simulink model "Third_order_loop"  (R2025a)
settings: Solver=VariableStepAuto  StartTime=0.0  StopTime=100  RelTol=1e-3
libraries: simulink x2
settings Model: Creator=庞亚宸  LastModifiedBy=庞亚宸

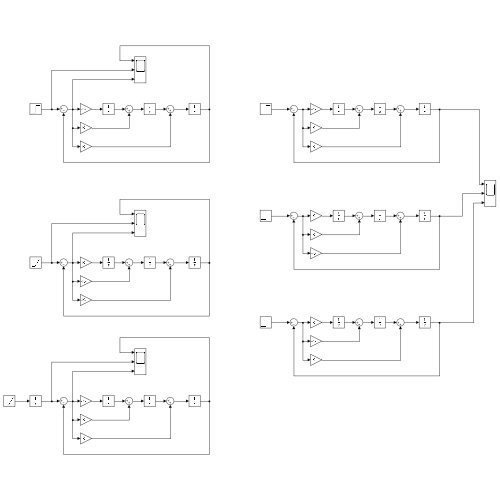
[thumbnail: Simulink's stored preview of the top-level diagram]
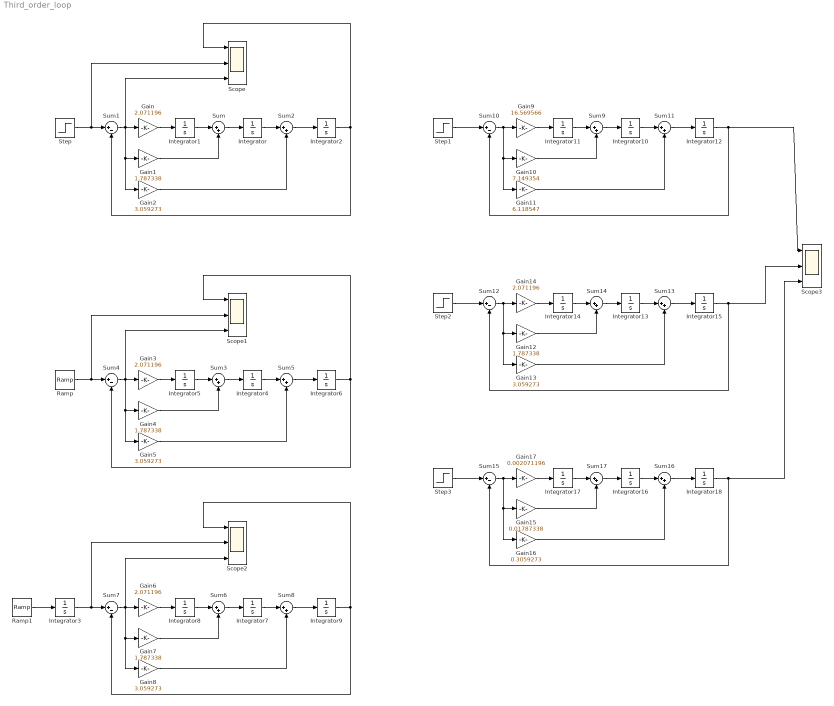
== system Third_order_loop ==
  Gain{,3,6,14} (4 alike) : Gain  Gain=2.071196
  Gain{1,4,7,12} (4 alike) : Gain  Gain=1.787338
  Gain10 : Gain  Gain=7.149354
  Gain11 : Gain  Gain=6.118547
  Gain{2,5,8,13} (4 alike) : Gain  Gain=3.059273
  Gain15 : Gain  Gain=0.01787338
  Gain16 : Gain  Gain=0.3059273
  Gain17 : Gain  Gain=0.002071196
  Gain9 : Gain  Gain=16.569566
  Integrator{,1..18} (19 alike) : Integrator
  Ramp : simulink/Sources/Ramp  slope=1  start=0  InitialOutput=0
  Ramp1 : simulink/Sources/Ramp  slope=1  start=0  InitialOutput=0
  Scope{,1..3} (4 alike) : Scope  NumInputPorts=3
      Scope settings: ActiveDisplayYMinimum=-0.15426727877104673  ActiveDisplayYMaximum=1.3884055089394209
      Scope1 settings: ActiveDisplayYMinimum=-12.500003189600191  ActiveDisplayYMaximum=112.50002870640175
      Scope2 settings: ActiveDisplayYMinimum=-624.99999881044585  ActiveDisplayYMaximum=5624.9999892940141  DataLoggingVariableName=ScopeData2
      Scope3 settings: ActiveDisplayYMinimum=-0.15460658948866587  ActiveDisplayYMaximum=1.3914593053979931  DataLoggingVariableName=ScopeData3
  Step{,1..3} (4 alike) : Step  Time=0  SampleTime=0
  Sum{,2..3,5..6,8..9,11,13..14,16..17} (12 alike) : Sum  Inputs=|++
  Sum{1,4,7,10,12,15} (6 alike) : Sum  Inputs=|+-
  wires:
  Sum/1 -> Integrator/1
  Gain/1 -> Integrator1/1
  Step/1 -> Scope/2, Sum1/1
  Sum1/1 -> Scope/3, Gain1/1, Gain2/1, Gain/1
  Ramp1/1 -> Integrator3/1
  Integrator1/1 -> Sum/1
  Gain1/1 -> Sum/2
  Integrator/1 -> Sum2/1
  Gain2/1 -> Sum2/2
  Sum2/1 -> Integrator2/1
  Integrator2/1 -> Sum1/2, Scope/1
  Integrator6/1 -> Sum4/2, Scope1/1
  Sum5/1 -> Integrator6/1
  Gain5/1 -> Sum5/2
  Sum3/1 -> Integrator4/1
  Gain4/1 -> Sum3/2
  Gain3/1 -> Integrator5/1
  Sum4/1 -> Scope1/3, Gain4/1, Gain5/1, Gain3/1
  Ramp/1 -> Scope1/2, Sum4/1
  Integrator5/1 -> Sum3/1
  Integrator4/1 -> Sum5/1
  Integrator9/1 -> Sum7/2, Scope2/1
  Sum8/1 -> Integrator9/1
  Gain8/1 -> Sum8/2
  Sum6/1 -> Integrator7/1
  Gain7/1 -> Sum6/2
  Gain6/1 -> Integrator8/1
  Sum7/1 -> Scope2/3, Gain7/1, Gain8/1, Gain6/1
  Integrator3/1 -> Scope2/2, Sum7/1
  Integrator8/1 -> Sum6/1
  Integrator7/1 -> Sum8/1
  Integrator12/1 -> Sum10/2, Scope3/1
  Sum11/1 -> Integrator12/1
  Gain11/1 -> Sum11/2
  Sum9/1 -> Integrator10/1
  Gain10/1 -> Sum9/2
  Gain9/1 -> Integrator11/1
  Sum10/1 -> Gain10/1, Gain11/1, Gain9/1
  Step1/1 -> Sum10/1
  Integrator11/1 -> Sum9/1
  Integrator10/1 -> Sum11/1
  Integrator13/1 -> Sum13/1
  Integrator14/1 -> Sum14/1
  Step2/1 -> Sum12/1
  Gain14/1 -> Integrator14/1
  Sum13/1 -> Integrator15/1
  Sum12/1 -> Gain12/1, Gain13/1, Gain14/1
  Sum14/1 -> Integrator13/1
  Gain12/1 -> Sum14/2
  Gain13/1 -> Sum13/2
  Integrator15/1 -> Scope3/2, Sum12/2
  Integrator16/1 -> Sum16/1
  Integrator17/1 -> Sum17/1
  Step3/1 -> Sum15/1
  Gain17/1 -> Integrator17/1
  Sum16/1 -> Integrator18/1
  Sum15/1 -> Gain15/1, Gain16/1, Gain17/1
  Sum17/1 -> Integrator16/1
  Gain15/1 -> Sum17/2
  Gain16/1 -> Sum16/2
  Integrator18/1 -> Scope3/3, Sum15/2
